simulink model "rolling_contact_36_example"  (R2026b)
settings: Solver=VariableStepAuto  StopTime=5
undefined symbols (not defined in the file): f_rr, k_gx, k_gy, k_x, m_wheel, miu_p, miu_s, mu_slide, mu_stick, omega_rr_eps, r_wheel, sgn, v_gx_max, v_gy_max, vLimit, X, Y, Z
libraries: nesl_utility x225, sm_lib x156, simulink x146, simulink_extras x36
(part 2 of 11)

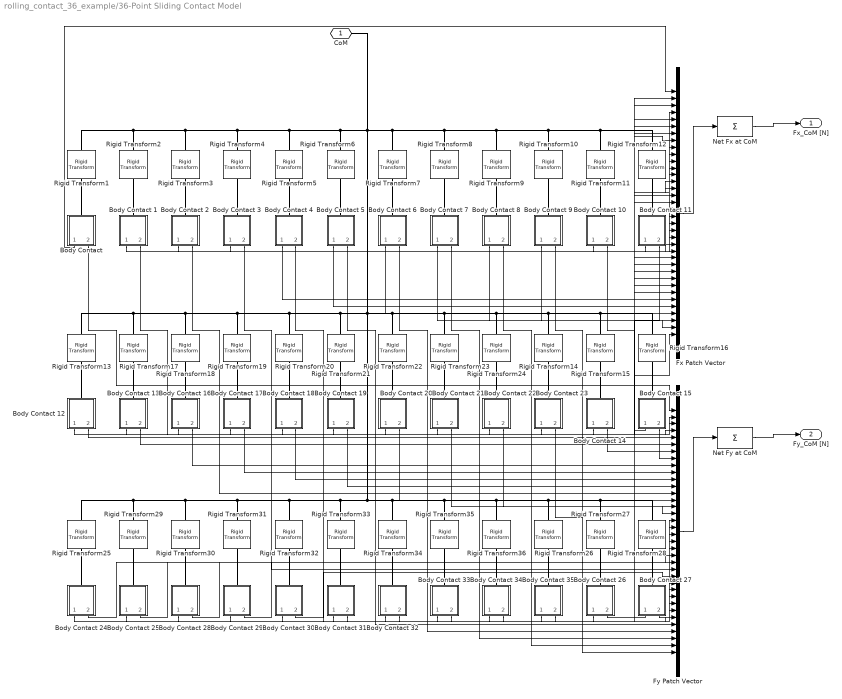
== system rolling_contact_36_example/36-Point Sliding Contact Model ==
  "Body Contact " : Subsystem
  Body Contact 1 : Subsystem
  Body Contact 10 : Subsystem
  Body Contact 11 : Subsystem
  Body Contact 12 : Subsystem
  Body Contact 13 : Subsystem
  Body Contact 14 : Subsystem
  Body Contact 15 : Subsystem
  Body Contact 16 : Subsystem
  Body Contact 17 : Subsystem
  Body Contact 18 : Subsystem
  Body Contact 19 : Subsystem
  Body Contact 2 : Subsystem
  Body Contact 20 : Subsystem
  Body Contact 21 : Subsystem
  Body Contact 22 : Subsystem
  Body Contact 23 : Subsystem
  Body Contact 24 : Subsystem
  Body Contact 25 : Subsystem
  Body Contact 26 : Subsystem
  Body Contact 27 : Subsystem
  Body Contact 28 : Subsystem
  Body Contact 29 : Subsystem
  Body Contact 3 : Subsystem
  Body Contact 30 : Subsystem
  Body Contact 31 : Subsystem
  Body Contact 32 : Subsystem
  Body Contact 33 : Subsystem
  Body Contact 34 : Subsystem
  Body Contact 35 : Subsystem
  Body Contact 4 : Subsystem
  Body Contact 5 : Subsystem
  Body Contact 6 : Subsystem
  Body Contact 7 : Subsystem
  Body Contact 8 : Subsystem
  Body Contact 9 : Subsystem
  Fx Patch Vector : Mux  Inputs=36
  Fy Patch Vector : Mux  Inputs=36
  Net Fx at CoM : Sum  Inputs=+
  Net Fy at CoM : Sum  Inputs=+
  Rigid Transform1 : sm_lib/Frames and Transforms/Rigid Transform  RotationMethod=None  FollAlignAxisA=+X  BaseAlignAxisA=+Y  FollAlignAxisB=+Y  BaseAlignAxisB=+Z  RotationStandardAxis=+Z  RotationAngle=0.0  RotationAngleUnits=deg  RotationArbitraryAxis=[0 0 1]  RotationSequenceAxes=FollowerAxes  RotationSequence=XYX  RotationSequenceAngles=[0 0 0]  RotationSequenceAnglesUnits=deg  RotationMatrix=[1 0 0; 0 1 0; 0 0 1]  Quaternion=[1 0 0 0]  TranslationMethod=Cylindrical  TranslationCartesianOffset=[0 0 0]  TranslationCartesianOffsetUnits=m  TranslationStandardAxis=+X  TranslationStandardOffset=+0.5  TranslationStandardOffsetUnits=m  TranslationROffset=r_ball  TranslationROffsetUnits=m  TranslationThetaOffset=0  TranslationThetaOffsetUnits=deg  TranslationZOffset=0  TranslationZOffsetUnits=m
  Rigid Transform10 : sm_lib/Frames and Transforms/Rigid Transform  RotationMethod=None  FollAlignAxisA=+X  BaseAlignAxisA=+Y  FollAlignAxisB=+Y  BaseAlignAxisB=+Z  RotationStandardAxis=+Z  RotationAngle=0.0  RotationAngleUnits=deg  RotationArbitraryAxis=[0 0 1]  RotationSequenceAxes=FollowerAxes  RotationSequence=XYX  RotationSequenceAngles=[0 0 0]  RotationSequenceAnglesUnits=deg  RotationMatrix=[1 0 0; 0 1 0; 0 0 1]  Quaternion=[1 0 0 0]  TranslationMethod=Cylindrical  TranslationCartesianOffset=[0 0 0]  TranslationCartesianOffsetUnits=m  TranslationStandardAxis=+X  TranslationStandardOffset=+0.5  TranslationStandardOffsetUnits=m  TranslationROffset=r_ball  TranslationROffsetUnits=m  TranslationThetaOffset=90  TranslationThetaOffsetUnits=deg  TranslationZOffset=0  TranslationZOffsetUnits=m
  Rigid Transform11 : sm_lib/Frames and Transforms/Rigid Transform  RotationMethod=None  FollAlignAxisA=+X  BaseAlignAxisA=+Y  FollAlignAxisB=+Y  BaseAlignAxisB=+Z  RotationStandardAxis=+Z  RotationAngle=0.0  RotationAngleUnits=deg  RotationArbitraryAxis=[0 0 1]  RotationSequenceAxes=FollowerAxes  RotationSequence=XYX  RotationSequenceAngles=[0 0 0]  RotationSequenceAnglesUnits=deg  RotationMatrix=[1 0 0; 0 1 0; 0 0 1]  Quaternion=[1 0 0 0]  TranslationMethod=Cylindrical  TranslationCartesianOffset=[0 0 0]  TranslationCartesianOffsetUnits=m  TranslationStandardAxis=+X  TranslationStandardOffset=+0.5  TranslationStandardOffsetUnits=m  TranslationROffset=r_ball  TranslationROffsetUnits=m  TranslationThetaOffset=100  TranslationThetaOffsetUnits=deg  TranslationZOffset=0  TranslationZOffsetUnits=m
  Rigid Transform12 : sm_lib/Frames and Transforms/Rigid Transform  RotationMethod=None  FollAlignAxisA=+X  BaseAlignAxisA=+Y  FollAlignAxisB=+Y  BaseAlignAxisB=+Z  RotationStandardAxis=+Z  RotationAngle=0.0  RotationAngleUnits=deg  RotationArbitraryAxis=[0 0 1]  RotationSequenceAxes=FollowerAxes  RotationSequence=XYX  RotationSequenceAngles=[0 0 0]  RotationSequenceAnglesUnits=deg  RotationMatrix=[1 0 0; 0 1 0; 0 0 1]  Quaternion=[1 0 0 0]  TranslationMethod=Cylindrical  TranslationCartesianOffset=[0 0 0]  TranslationCartesianOffsetUnits=m  TranslationStandardAxis=+X  TranslationStandardOffset=+0.5  TranslationStandardOffsetUnits=m  TranslationROffset=r_ball  TranslationROffsetUnits=m  TranslationThetaOffset=110  TranslationThetaOffsetUnits=deg  TranslationZOffset=0  TranslationZOffsetUnits=m
  Rigid Transform13 : sm_lib/Frames and Transforms/Rigid Transform  RotationMethod=None  FollAlignAxisA=+X  BaseAlignAxisA=+Y  FollAlignAxisB=+Y  BaseAlignAxisB=+Z  RotationStandardAxis=+Z  RotationAngle=0.0  RotationAngleUnits=deg  RotationArbitraryAxis=[0 0 1]  RotationSequenceAxes=FollowerAxes  RotationSequence=XYX  RotationSequenceAngles=[0 0 0]  RotationSequenceAnglesUnits=deg  RotationMatrix=[1 0 0; 0 1 0; 0 0 1]  Quaternion=[1 0 0 0]  TranslationMethod=Cylindrical  TranslationCartesianOffset=[0 0 0]  TranslationCartesianOffsetUnits=m  TranslationStandardAxis=+X  TranslationStandardOffset=+0.5  TranslationStandardOffsetUnits=m  TranslationROffset=r_ball  TranslationROffsetUnits=m  TranslationThetaOffset=120  TranslationThetaOffsetUnits=deg  TranslationZOffset=0  TranslationZOffsetUnits=m
  Rigid Transform14 : sm_lib/Frames and Transforms/Rigid Transform  RotationMethod=None  FollAlignAxisA=+X  BaseAlignAxisA=+Y  FollAlignAxisB=+Y  BaseAlignAxisB=+Z  RotationStandardAxis=+Z  RotationAngle=0.0  RotationAngleUnits=deg  RotationArbitraryAxis=[0 0 1]  RotationSequenceAxes=FollowerAxes  RotationSequence=XYX  RotationSequenceAngles=[0 0 0]  RotationSequenceAnglesUnits=deg  RotationMatrix=[1 0 0; 0 1 0; 0 0 1]  Quaternion=[1 0 0 0]  TranslationMethod=Cylindrical  TranslationCartesianOffset=[0 0 0]  TranslationCartesianOffsetUnits=m  TranslationStandardAxis=+X  TranslationStandardOffset=+0.5  TranslationStandardOffsetUnits=m  TranslationROffset=r_ball  TranslationROffsetUnits=m  TranslationThetaOffset=210  TranslationThetaOffsetUnits=deg  TranslationZOffset=0  TranslationZOffsetUnits=m
  Rigid Transform15 : sm_lib/Frames and Transforms/Rigid Transform  RotationMethod=None  FollAlignAxisA=+X  BaseAlignAxisA=+Y  FollAlignAxisB=+Y  BaseAlignAxisB=+Z  RotationStandardAxis=+Z  RotationAngle=0.0  RotationAngleUnits=deg  RotationArbitraryAxis=[0 0 1]  RotationSequenceAxes=FollowerAxes  RotationSequence=XYX  RotationSequenceAngles=[0 0 0]  RotationSequenceAnglesUnits=deg  RotationMatrix=[1 0 0; 0 1 0; 0 0 1]  Quaternion=[1 0 0 0]  TranslationMethod=Cylindrical  TranslationCartesianOffset=[0 0 0]  TranslationCartesianOffsetUnits=m  TranslationStandardAxis=+X  TranslationStandardOffset=+0.5  TranslationStandardOffsetUnits=m  TranslationROffset=r_ball  TranslationROffsetUnits=m  TranslationThetaOffset=220  TranslationThetaOffsetUnits=deg  TranslationZOffset=0  TranslationZOffsetUnits=m
  Rigid Transform16 : sm_lib/Frames and Transforms/Rigid Transform  RotationMethod=None  FollAlignAxisA=+X  BaseAlignAxisA=+Y  FollAlignAxisB=+Y  BaseAlignAxisB=+Z  RotationStandardAxis=+Z  RotationAngle=0.0  RotationAngleUnits=deg  RotationArbitraryAxis=[0 0 1]  RotationSequenceAxes=FollowerAxes  RotationSequence=XYX  RotationSequenceAngles=[0 0 0]  RotationSequenceAnglesUnits=deg  RotationMatrix=[1 0 0; 0 1 0; 0 0 1]  Quaternion=[1 0 0 0]  TranslationMethod=Cylindrical  TranslationCartesianOffset=[0 0 0]  TranslationCartesianOffsetUnits=m  TranslationStandardAxis=+X  TranslationStandardOffset=+0.5  TranslationStandardOffsetUnits=m  TranslationROffset=r_ball  TranslationROffsetUnits=m  TranslationThetaOffset=230  TranslationThetaOffsetUnits=deg  TranslationZOffset=0  TranslationZOffsetUnits=m
  Rigid Transform17 : sm_lib/Frames and Transforms/Rigid Transform  RotationMethod=None  FollAlignAxisA=+X  BaseAlignAxisA=+Y  FollAlignAxisB=+Y  BaseAlignAxisB=+Z  RotationStandardAxis=+Z  RotationAngle=0.0  RotationAngleUnits=deg  RotationArbitraryAxis=[0 0 1]  RotationSequenceAxes=FollowerAxes  RotationSequence=XYX  RotationSequenceAngles=[0 0 0]  RotationSequenceAnglesUnits=deg  RotationMatrix=[1 0 0; 0 1 0; 0 0 1]  Quaternion=[1 0 0 0]  TranslationMethod=Cylindrical  TranslationCartesianOffset=[0 0 0]  TranslationCartesianOffsetUnits=m  TranslationStandardAxis=+X  TranslationStandardOffset=+0.5  TranslationStandardOffsetUnits=m  TranslationROffset=r_ball  TranslationROffsetUnits=m  TranslationThetaOffset=130  TranslationThetaOffsetUnits=deg  TranslationZOffset=0  TranslationZOffsetUnits=m
  Rigid Transform18 : sm_lib/Frames and Transforms/Rigid Transform  RotationMethod=None  FollAlignAxisA=+X  BaseAlignAxisA=+Y  FollAlignAxisB=+Y  BaseAlignAxisB=+Z  RotationStandardAxis=+Z  RotationAngle=0.0  RotationAngleUnits=deg  RotationArbitraryAxis=[0 0 1]  RotationSequenceAxes=FollowerAxes  RotationSequence=XYX  RotationSequenceAngles=[0 0 0]  RotationSequenceAnglesUnits=deg  RotationMatrix=[1 0 0; 0 1 0; 0 0 1]  Quaternion=[1 0 0 0]  TranslationMethod=Cylindrical  TranslationCartesianOffset=[0 0 0]  TranslationCartesianOffsetUnits=m  TranslationStandardAxis=+X  TranslationStandardOffset=+0.5  TranslationStandardOffsetUnits=m  TranslationROffset=r_ball  TranslationROffsetUnits=m  TranslationThetaOffset=140  TranslationThetaOffsetUnits=deg  TranslationZOffset=0  TranslationZOffsetUnits=m
  Rigid Transform19 : sm_lib/Frames and Transforms/Rigid Transform  RotationMethod=None  FollAlignAxisA=+X  BaseAlignAxisA=+Y  FollAlignAxisB=+Y  BaseAlignAxisB=+Z  RotationStandardAxis=+Z  RotationAngle=0.0  RotationAngleUnits=deg  RotationArbitraryAxis=[0 0 1]  RotationSequenceAxes=FollowerAxes  RotationSequence=XYX  RotationSequenceAngles=[0 0 0]  RotationSequenceAnglesUnits=deg  RotationMatrix=[1 0 0; 0 1 0; 0 0 1]  Quaternion=[1 0 0 0]  TranslationMethod=Cylindrical  TranslationCartesianOffset=[0 0 0]  TranslationCartesianOffsetUnits=m  TranslationStandardAxis=+X  TranslationStandardOffset=+0.5  TranslationStandardOffsetUnits=m  TranslationROffset=r_ball  TranslationROffsetUnits=m  TranslationThetaOffset=150  TranslationThetaOffsetUnits=deg  TranslationZOffset=0  TranslationZOffsetUnits=m
  Rigid Transform2 : sm_lib/Frames and Transforms/Rigid Transform  RotationMethod=None  FollAlignAxisA=+X  BaseAlignAxisA=+Y  FollAlignAxisB=+Y  BaseAlignAxisB=+Z  RotationStandardAxis=+Z  RotationAngle=0.0  RotationAngleUnits=deg  RotationArbitraryAxis=[0 0 1]  RotationSequenceAxes=FollowerAxes  RotationSequence=XYX  RotationSequenceAngles=[0 0 0]  RotationSequenceAnglesUnits=deg  RotationMatrix=[1 0 0; 0 1 0; 0 0 1]  Quaternion=[1 0 0 0]  TranslationMethod=Cylindrical  TranslationCartesianOffset=[0 0 0]  TranslationCartesianOffsetUnits=m  TranslationStandardAxis=+X  TranslationStandardOffset=+0.5  TranslationStandardOffsetUnits=m  TranslationROffset=r_ball  TranslationROffsetUnits=m  TranslationThetaOffset=10  TranslationThetaOffsetUnits=deg  TranslationZOffset=0  TranslationZOffsetUnits=m
  Rigid Transform20 : sm_lib/Frames and Transforms/Rigid Transform  RotationMethod=None  FollAlignAxisA=+X  BaseAlignAxisA=+Y  FollAlignAxisB=+Y  BaseAlignAxisB=+Z  RotationStandardAxis=+Z  RotationAngle=0.0  RotationAngleUnits=deg  RotationArbitraryAxis=[0 0 1]  RotationSequenceAxes=FollowerAxes  RotationSequence=XYX  RotationSequenceAngles=[0 0 0]  RotationSequenceAnglesUnits=deg  RotationMatrix=[1 0 0; 0 1 0; 0 0 1]  Quaternion=[1 0 0 0]  TranslationMethod=Cylindrical  TranslationCartesianOffset=[0 0 0]  TranslationCartesianOffsetUnits=m  TranslationStandardAxis=+X  TranslationStandardOffset=+0.5  TranslationStandardOffsetUnits=m  TranslationROffset=r_ball  TranslationROffsetUnits=m  TranslationThetaOffset=160  TranslationThetaOffsetUnits=deg  TranslationZOffset=0  TranslationZOffsetUnits=m
  Rigid Transform21 : sm_lib/Frames and Transforms/Rigid Transform  RotationMethod=None  FollAlignAxisA=+X  BaseAlignAxisA=+Y  FollAlignAxisB=+Y  BaseAlignAxisB=+Z  RotationStandardAxis=+Z  RotationAngle=0.0  RotationAngleUnits=deg  RotationArbitraryAxis=[0 0 1]  RotationSequenceAxes=FollowerAxes  RotationSequence=XYX  RotationSequenceAngles=[0 0 0]  RotationSequenceAnglesUnits=deg  RotationMatrix=[1 0 0; 0 1 0; 0 0 1]  Quaternion=[1 0 0 0]  TranslationMethod=Cylindrical  TranslationCartesianOffset=[0 0 0]  TranslationCartesianOffsetUnits=m  TranslationStandardAxis=+X  TranslationStandardOffset=+0.5  TranslationStandardOffsetUnits=m  TranslationROffset=r_ball  TranslationROffsetUnits=m  TranslationThetaOffset=170  TranslationThetaOffsetUnits=deg  TranslationZOffset=0  TranslationZOffsetUnits=m
  Rigid Transform22 : sm_lib/Frames and Transforms/Rigid Transform  RotationMethod=None  FollAlignAxisA=+X  BaseAlignAxisA=+Y  FollAlignAxisB=+Y  BaseAlignAxisB=+Z  RotationStandardAxis=+Z  RotationAngle=0.0  RotationAngleUnits=deg  RotationArbitraryAxis=[0 0 1]  RotationSequenceAxes=FollowerAxes  RotationSequence=XYX  RotationSequenceAngles=[0 0 0]  RotationSequenceAnglesUnits=deg  RotationMatrix=[1 0 0; 0 1 0; 0 0 1]  Quaternion=[1 0 0 0]  TranslationMethod=Cylindrical  TranslationCartesianOffset=[0 0 0]  TranslationCartesianOffsetUnits=m  TranslationStandardAxis=+X  TranslationStandardOffset=+0.5  TranslationStandardOffsetUnits=m  TranslationROffset=r_ball  TranslationROffsetUnits=m  TranslationThetaOffset=180  TranslationThetaOffsetUnits=deg  TranslationZOffset=0  TranslationZOffsetUnits=m
  Rigid Transform23 : sm_lib/Frames and Transforms/Rigid Transform  RotationMethod=None  FollAlignAxisA=+X  BaseAlignAxisA=+Y  FollAlignAxisB=+Y  BaseAlignAxisB=+Z  RotationStandardAxis=+Z  RotationAngle=0.0  RotationAngleUnits=deg  RotationArbitraryAxis=[0 0 1]  RotationSequenceAxes=FollowerAxes  RotationSequence=XYX  RotationSequenceAngles=[0 0 0]  RotationSequenceAnglesUnits=deg  RotationMatrix=[1 0 0; 0 1 0; 0 0 1]  Quaternion=[1 0 0 0]  TranslationMethod=Cylindrical  TranslationCartesianOffset=[0 0 0]  TranslationCartesianOffsetUnits=m  TranslationStandardAxis=+X  TranslationStandardOffset=+0.5  TranslationStandardOffsetUnits=m  TranslationROffset=r_ball  TranslationROffsetUnits=m  TranslationThetaOffset=190  TranslationThetaOffsetUnits=deg  TranslationZOffset=0  TranslationZOffsetUnits=m
  Rigid Transform24 : sm_lib/Frames and Transforms/Rigid Transform  RotationMethod=None  FollAlignAxisA=+X  BaseAlignAxisA=+Y  FollAlignAxisB=+Y  BaseAlignAxisB=+Z  RotationStandardAxis=+Z  RotationAngle=0.0  RotationAngleUnits=deg  RotationArbitraryAxis=[0 0 1]  RotationSequenceAxes=FollowerAxes  RotationSequence=XYX  RotationSequenceAngles=[0 0 0]  RotationSequenceAnglesUnits=deg  RotationMatrix=[1 0 0; 0 1 0; 0 0 1]  Quaternion=[1 0 0 0]  TranslationMethod=Cylindrical  TranslationCartesianOffset=[0 0 0]  TranslationCartesianOffsetUnits=m  TranslationStandardAxis=+X  TranslationStandardOffset=+0.5  TranslationStandardOffsetUnits=m  TranslationROffset=r_ball  TranslationROffsetUnits=m  TranslationThetaOffset=200  TranslationThetaOffsetUnits=deg  TranslationZOffset=0  TranslationZOffsetUnits=m
  Rigid Transform25 : sm_lib/Frames and Transforms/Rigid Transform  RotationMethod=None  FollAlignAxisA=+X  BaseAlignAxisA=+Y  FollAlignAxisB=+Y  BaseAlignAxisB=+Z  RotationStandardAxis=+Z  RotationAngle=0.0  RotationAngleUnits=deg  RotationArbitraryAxis=[0 0 1]  RotationSequenceAxes=FollowerAxes  RotationSequence=XYX  RotationSequenceAngles=[0 0 0]  RotationSequenceAnglesUnits=deg  RotationMatrix=[1 0 0; 0 1 0; 0 0 1]  Quaternion=[1 0 0 0]  TranslationMethod=Cylindrical  TranslationCartesianOffset=[0 0 0]  TranslationCartesianOffsetUnits=m  TranslationStandardAxis=+X  TranslationStandardOffset=+0.5  TranslationStandardOffsetUnits=m  TranslationROffset=r_ball  TranslationROffsetUnits=m  TranslationThetaOffset=240  TranslationThetaOffsetUnits=deg  TranslationZOffset=0  TranslationZOffsetUnits=m
  Rigid Transform26 : sm_lib/Frames and Transforms/Rigid Transform  RotationMethod=None  FollAlignAxisA=+X  BaseAlignAxisA=+Y  FollAlignAxisB=+Y  BaseAlignAxisB=+Z  RotationStandardAxis=+Z  RotationAngle=0.0  RotationAngleUnits=deg  RotationArbitraryAxis=[0 0 1]  RotationSequenceAxes=FollowerAxes  RotationSequence=XYX  RotationSequenceAngles=[0 0 0]  RotationSequenceAnglesUnits=deg  RotationMatrix=[1 0 0; 0 1 0; 0 0 1]  Quaternion=[1 0 0 0]  TranslationMethod=Cylindrical  TranslationCartesianOffset=[0 0 0]  TranslationCartesianOffsetUnits=m  TranslationStandardAxis=+X  TranslationStandardOffset=+0.5  TranslationStandardOffsetUnits=m  TranslationROffset=r_ball  TranslationROffsetUnits=m  TranslationThetaOffset=330  TranslationThetaOffsetUnits=deg  TranslationZOffset=0  TranslationZOffsetUnits=m
  Rigid Transform27 : sm_lib/Frames and Transforms/Rigid Transform  RotationMethod=None  FollAlignAxisA=+X  BaseAlignAxisA=+Y  FollAlignAxisB=+Y  BaseAlignAxisB=+Z  RotationStandardAxis=+Z  RotationAngle=0.0  RotationAngleUnits=deg  RotationArbitraryAxis=[0 0 1]  RotationSequenceAxes=FollowerAxes  RotationSequence=XYX  RotationSequenceAngles=[0 0 0]  RotationSequenceAnglesUnits=deg  RotationMatrix=[1 0 0; 0 1 0; 0 0 1]  Quaternion=[1 0 0 0]  TranslationMethod=Cylindrical  TranslationCartesianOffset=[0 0 0]  TranslationCartesianOffsetUnits=m  TranslationStandardAxis=+X  TranslationStandardOffset=+0.5  TranslationStandardOffsetUnits=m  TranslationROffset=r_ball  TranslationROffsetUnits=m  TranslationThetaOffset=340  TranslationThetaOffsetUnits=deg  TranslationZOffset=0  TranslationZOffsetUnits=m
  Rigid Transform28 : sm_lib/Frames and Transforms/Rigid Transform  RotationMethod=None  FollAlignAxisA=+X  BaseAlignAxisA=+Y  FollAlignAxisB=+Y  BaseAlignAxisB=+Z  RotationStandardAxis=+Z  RotationAngle=0.0  RotationAngleUnits=deg  RotationArbitraryAxis=[0 0 1]  RotationSequenceAxes=FollowerAxes  RotationSequence=XYX  RotationSequenceAngles=[0 0 0]  RotationSequenceAnglesUnits=deg  RotationMatrix=[1 0 0; 0 1 0; 0 0 1]  Quaternion=[1 0 0 0]  TranslationMethod=Cylindrical  TranslationCartesianOffset=[0 0 0]  TranslationCartesianOffsetUnits=m  TranslationStandardAxis=+X  TranslationStandardOffset=+0.5  TranslationStandardOffsetUnits=m  TranslationROffset=r_ball  TranslationROffsetUnits=m  TranslationThetaOffset=350  TranslationThetaOffsetUnits=deg  TranslationZOffset=0  TranslationZOffsetUnits=m
  Rigid Transform29 : sm_lib/Frames and Transforms/Rigid Transform  RotationMethod=None  FollAlignAxisA=+X  BaseAlignAxisA=+Y  FollAlignAxisB=+Y  BaseAlignAxisB=+Z  RotationStandardAxis=+Z  RotationAngle=0.0  RotationAngleUnits=deg  RotationArbitraryAxis=[0 0 1]  RotationSequenceAxes=FollowerAxes  RotationSequence=XYX  RotationSequenceAngles=[0 0 0]  RotationSequenceAnglesUnits=deg  RotationMatrix=[1 0 0; 0 1 0; 0 0 1]  Quaternion=[1 0 0 0]  TranslationMethod=Cylindrical  TranslationCartesianOffset=[0 0 0]  TranslationCartesianOffsetUnits=m  TranslationStandardAxis=+X  TranslationStandardOffset=+0.5  TranslationStandardOffsetUnits=m  TranslationROffset=r_ball  TranslationROffsetUnits=m  TranslationThetaOffset=250  TranslationThetaOffsetUnits=deg  TranslationZOffset=0  TranslationZOffsetUnits=m
  Rigid Transform3 : sm_lib/Frames and Transforms/Rigid Transform  RotationMethod=None  FollAlignAxisA=+X  BaseAlignAxisA=+Y  FollAlignAxisB=+Y  BaseAlignAxisB=+Z  RotationStandardAxis=+Z  RotationAngle=0.0  RotationAngleUnits=deg  RotationArbitraryAxis=[0 0 1]  RotationSequenceAxes=FollowerAxes  RotationSequence=XYX  RotationSequenceAngles=[0 0 0]  RotationSequenceAnglesUnits=deg  RotationMatrix=[1 0 0; 0 1 0; 0 0 1]  Quaternion=[1 0 0 0]  TranslationMethod=Cylindrical  TranslationCartesianOffset=[0 0 0]  TranslationCartesianOffsetUnits=m  TranslationStandardAxis=+X  TranslationStandardOffset=+0.5  TranslationStandardOffsetUnits=m  TranslationROffset=r_ball  TranslationROffsetUnits=m  TranslationThetaOffset=20  TranslationThetaOffsetUnits=deg  TranslationZOffset=0  TranslationZOffsetUnits=m
  Rigid Transform30 : sm_lib/Frames and Transforms/Rigid Transform  RotationMethod=None  FollAlignAxisA=+X  BaseAlignAxisA=+Y  FollAlignAxisB=+Y  BaseAlignAxisB=+Z  RotationStandardAxis=+Z  RotationAngle=0.0  RotationAngleUnits=deg  RotationArbitraryAxis=[0 0 1]  RotationSequenceAxes=FollowerAxes  RotationSequence=XYX  RotationSequenceAngles=[0 0 0]  RotationSequenceAnglesUnits=deg  RotationMatrix=[1 0 0; 0 1 0; 0 0 1]  Quaternion=[1 0 0 0]  TranslationMethod=Cylindrical  TranslationCartesianOffset=[0 0 0]  TranslationCartesianOffsetUnits=m  TranslationStandardAxis=+X  TranslationStandardOffset=+0.5  TranslationStandardOffsetUnits=m  TranslationROffset=r_ball  TranslationROffsetUnits=m  TranslationThetaOffset=260  TranslationThetaOffsetUnits=deg  TranslationZOffset=0  TranslationZOffsetUnits=m
  Rigid Transform31 : sm_lib/Frames and Transforms/Rigid Transform  RotationMethod=None  FollAlignAxisA=+X  BaseAlignAxisA=+Y  FollAlignAxisB=+Y  BaseAlignAxisB=+Z  RotationStandardAxis=+Z  RotationAngle=0.0  RotationAngleUnits=deg  RotationArbitraryAxis=[0 0 1]  RotationSequenceAxes=FollowerAxes  RotationSequence=XYX  RotationSequenceAngles=[0 0 0]  RotationSequenceAnglesUnits=deg  RotationMatrix=[1 0 0; 0 1 0; 0 0 1]  Quaternion=[1 0 0 0]  TranslationMethod=Cylindrical  TranslationCartesianOffset=[0 0 0]  TranslationCartesianOffsetUnits=m  TranslationStandardAxis=+X  TranslationStandardOffset=+0.5  TranslationStandardOffsetUnits=m  TranslationROffset=r_ball  TranslationROffsetUnits=m  TranslationThetaOffset=270  TranslationThetaOffsetUnits=deg  TranslationZOffset=0  TranslationZOffsetUnits=m
  Rigid Transform32 : sm_lib/Frames and Transforms/Rigid Transform  RotationMethod=None  FollAlignAxisA=+X  BaseAlignAxisA=+Y  FollAlignAxisB=+Y  BaseAlignAxisB=+Z  RotationStandardAxis=+Z  RotationAngle=0.0  RotationAngleUnits=deg  RotationArbitraryAxis=[0 0 1]  RotationSequenceAxes=FollowerAxes  RotationSequence=XYX  RotationSequenceAngles=[0 0 0]  RotationSequenceAnglesUnits=deg  RotationMatrix=[1 0 0; 0 1 0; 0 0 1]  Quaternion=[1 0 0 0]  TranslationMethod=Cylindrical  TranslationCartesianOffset=[0 0 0]  TranslationCartesianOffsetUnits=m  TranslationStandardAxis=+X  TranslationStandardOffset=+0.5  TranslationStandardOffsetUnits=m  TranslationROffset=r_ball  TranslationROffsetUnits=m  TranslationThetaOffset=280  TranslationThetaOffsetUnits=deg  TranslationZOffset=0  TranslationZOffsetUnits=m
  Rigid Transform33 : sm_lib/Frames and Transforms/Rigid Transform  RotationMethod=None  FollAlignAxisA=+X  BaseAlignAxisA=+Y  FollAlignAxisB=+Y  BaseAlignAxisB=+Z  RotationStandardAxis=+Z  RotationAngle=0.0  RotationAngleUnits=deg  RotationArbitraryAxis=[0 0 1]  RotationSequenceAxes=FollowerAxes  RotationSequence=XYX  RotationSequenceAngles=[0 0 0]  RotationSequenceAnglesUnits=deg  RotationMatrix=[1 0 0; 0 1 0; 0 0 1]  Quaternion=[1 0 0 0]  TranslationMethod=Cylindrical  TranslationCartesianOffset=[0 0 0]  TranslationCartesianOffsetUnits=m  TranslationStandardAxis=+X  TranslationStandardOffset=+0.5  TranslationStandardOffsetUnits=m  TranslationROffset=r_ball  TranslationROffsetUnits=m  TranslationThetaOffset=290  TranslationThetaOffsetUnits=deg  TranslationZOffset=0  TranslationZOffsetUnits=m
  Rigid Transform34 : sm_lib/Frames and Transforms/Rigid Transform  RotationMethod=None  FollAlignAxisA=+X  BaseAlignAxisA=+Y  FollAlignAxisB=+Y  BaseAlignAxisB=+Z  RotationStandardAxis=+Z  RotationAngle=0.0  RotationAngleUnits=deg  RotationArbitraryAxis=[0 0 1]  RotationSequenceAxes=FollowerAxes  RotationSequence=XYX  RotationSequenceAngles=[0 0 0]  RotationSequenceAnglesUnits=deg  RotationMatrix=[1 0 0; 0 1 0; 0 0 1]  Quaternion=[1 0 0 0]  TranslationMethod=Cylindrical  TranslationCartesianOffset=[0 0 0]  TranslationCartesianOffsetUnits=m  TranslationStandardAxis=+X  TranslationStandardOffset=+0.5  TranslationStandardOffsetUnits=m  TranslationROffset=r_ball  TranslationROffsetUnits=m  TranslationThetaOffset=300  TranslationThetaOffsetUnits=deg  TranslationZOffset=0  TranslationZOffsetUnits=m
  Rigid Transform35 : sm_lib/Frames and Transforms/Rigid Transform  RotationMethod=None  FollAlignAxisA=+X  BaseAlignAxisA=+Y  FollAlignAxisB=+Y  BaseAlignAxisB=+Z  RotationStandardAxis=+Z  RotationAngle=0.0  RotationAngleUnits=deg  RotationArbitraryAxis=[0 0 1]  RotationSequenceAxes=FollowerAxes  RotationSequence=XYX  RotationSequenceAngles=[0 0 0]  RotationSequenceAnglesUnits=deg  RotationMatrix=[1 0 0; 0 1 0; 0 0 1]  Quaternion=[1 0 0 0]  TranslationMethod=Cylindrical  TranslationCartesianOffset=[0 0 0]  TranslationCartesianOffsetUnits=m  TranslationStandardAxis=+X  TranslationStandardOffset=+0.5  TranslationStandardOffsetUnits=m  TranslationROffset=r_ball  TranslationROffsetUnits=m  TranslationThetaOffset=310  TranslationThetaOffsetUnits=deg  TranslationZOffset=0  TranslationZOffsetUnits=m
  Rigid Transform36 : sm_lib/Frames and Transforms/Rigid Transform  RotationMethod=None  FollAlignAxisA=+X  BaseAlignAxisA=+Y  FollAlignAxisB=+Y  BaseAlignAxisB=+Z  RotationStandardAxis=+Z  RotationAngle=0.0  RotationAngleUnits=deg  RotationArbitraryAxis=[0 0 1]  RotationSequenceAxes=FollowerAxes  RotationSequence=XYX  RotationSequenceAngles=[0 0 0]  RotationSequenceAnglesUnits=deg  RotationMatrix=[1 0 0; 0 1 0; 0 0 1]  Quaternion=[1 0 0 0]  TranslationMethod=Cylindrical  TranslationCartesianOffset=[0 0 0]  TranslationCartesianOffsetUnits=m  TranslationStandardAxis=+X  TranslationStandardOffset=+0.5  TranslationStandardOffsetUnits=m  TranslationROffset=r_ball  TranslationROffsetUnits=m  TranslationThetaOffset=320  TranslationThetaOffsetUnits=deg  TranslationZOffset=0  TranslationZOffsetUnits=m
  Rigid Transform4 : sm_lib/Frames and Transforms/Rigid Transform  RotationMethod=None  FollAlignAxisA=+X  BaseAlignAxisA=+Y  FollAlignAxisB=+Y  BaseAlignAxisB=+Z  RotationStandardAxis=+Z  RotationAngle=0.0  RotationAngleUnits=deg  RotationArbitraryAxis=[0 0 1]  RotationSequenceAxes=FollowerAxes  RotationSequence=XYX  RotationSequenceAngles=[0 0 0]  RotationSequenceAnglesUnits=deg  RotationMatrix=[1 0 0; 0 1 0; 0 0 1]  Quaternion=[1 0 0 0]  TranslationMethod=Cylindrical  TranslationCartesianOffset=[0 0 0]  TranslationCartesianOffsetUnits=m  TranslationStandardAxis=+X  TranslationStandardOffset=+0.5  TranslationStandardOffsetUnits=m  TranslationROffset=r_ball  TranslationROffsetUnits=m  TranslationThetaOffset=30  TranslationThetaOffsetUnits=deg  TranslationZOffset=0  TranslationZOffsetUnits=m
  Rigid Transform5 : sm_lib/Frames and Transforms/Rigid Transform  RotationMethod=None  FollAlignAxisA=+X  BaseAlignAxisA=+Y  FollAlignAxisB=+Y  BaseAlignAxisB=+Z  RotationStandardAxis=+Z  RotationAngle=0.0  RotationAngleUnits=deg  RotationArbitraryAxis=[0 0 1]  RotationSequenceAxes=FollowerAxes  RotationSequence=XYX  RotationSequenceAngles=[0 0 0]  RotationSequenceAnglesUnits=deg  RotationMatrix=[1 0 0; 0 1 0; 0 0 1]  Quaternion=[1 0 0 0]  TranslationMethod=Cylindrical  TranslationCartesianOffset=[0 0 0]  TranslationCartesianOffsetUnits=m  TranslationStandardAxis=+X  TranslationStandardOffset=+0.5  TranslationStandardOffsetUnits=m  TranslationROffset=r_ball  TranslationROffsetUnits=m  TranslationThetaOffset=40  TranslationThetaOffsetUnits=deg  TranslationZOffset=0  TranslationZOffsetUnits=m
  Rigid Transform6 : sm_lib/Frames and Transforms/Rigid Transform  RotationMethod=None  FollAlignAxisA=+X  BaseAlignAxisA=+Y  FollAlignAxisB=+Y  BaseAlignAxisB=+Z  RotationStandardAxis=+Z  RotationAngle=0.0  RotationAngleUnits=deg  RotationArbitraryAxis=[0 0 1]  RotationSequenceAxes=FollowerAxes  RotationSequence=XYX  RotationSequenceAngles=[0 0 0]  RotationSequenceAnglesUnits=deg  RotationMatrix=[1 0 0; 0 1 0; 0 0 1]  Quaternion=[1 0 0 0]  TranslationMethod=Cylindrical  TranslationCartesianOffset=[0 0 0]  TranslationCartesianOffsetUnits=m  TranslationStandardAxis=+X  TranslationStandardOffset=+0.5  TranslationStandardOffsetUnits=m  TranslationROffset=r_ball  TranslationROffsetUnits=m  TranslationThetaOffset=50  TranslationThetaOffsetUnits=deg  TranslationZOffset=0  TranslationZOffsetUnits=m
  Rigid Transform7 : sm_lib/Frames and Transforms/Rigid Transform  RotationMethod=None  FollAlignAxisA=+X  BaseAlignAxisA=+Y  FollAlignAxisB=+Y  BaseAlignAxisB=+Z  RotationStandardAxis=+Z  RotationAngle=0.0  RotationAngleUnits=deg  RotationArbitraryAxis=[0 0 1]  RotationSequenceAxes=FollowerAxes  RotationSequence=XYX  RotationSequenceAngles=[0 0 0]  RotationSequenceAnglesUnits=deg  RotationMatrix=[1 0 0; 0 1 0; 0 0 1]  Quaternion=[1 0 0 0]  TranslationMethod=Cylindrical  TranslationCartesianOffset=[0 0 0]  TranslationCartesianOffsetUnits=m  TranslationStandardAxis=+X  TranslationStandardOffset=+0.5  TranslationStandardOffsetUnits=m  TranslationROffset=r_ball  TranslationROffsetUnits=m  TranslationThetaOffset=60  TranslationThetaOffsetUnits=deg  TranslationZOffset=0  TranslationZOffsetUnits=m
  Rigid Transform8 : sm_lib/Frames and Transforms/Rigid Transform  RotationMethod=None  FollAlignAxisA=+X  BaseAlignAxisA=+Y  FollAlignAxisB=+Y  BaseAlignAxisB=+Z  RotationStandardAxis=+Z  RotationAngle=0.0  RotationAngleUnits=deg  RotationArbitraryAxis=[0 0 1]  RotationSequenceAxes=FollowerAxes  RotationSequence=XYX  RotationSequenceAngles=[0 0 0]  RotationSequenceAnglesUnits=deg  RotationMatrix=[1 0 0; 0 1 0; 0 0 1]  Quaternion=[1 0 0 0]  TranslationMethod=Cylindrical  TranslationCartesianOffset=[0 0 0]  TranslationCartesianOffsetUnits=m  TranslationStandardAxis=+X  TranslationStandardOffset=+0.5  TranslationStandardOffsetUnits=m  TranslationROffset=r_ball  TranslationROffsetUnits=m  TranslationThetaOffset=70  TranslationThetaOffsetUnits=deg  TranslationZOffset=0  TranslationZOffsetUnits=m
  Rigid Transform9 : sm_lib/Frames and Transforms/Rigid Transform  RotationMethod=None  FollAlignAxisA=+X  BaseAlignAxisA=+Y  FollAlignAxisB=+Y  BaseAlignAxisB=+Z  RotationStandardAxis=+Z  RotationAngle=0.0  RotationAngleUnits=deg  RotationArbitraryAxis=[0 0 1]  RotationSequenceAxes=FollowerAxes  RotationSequence=XYX  RotationSequenceAngles=[0 0 0]  RotationSequenceAnglesUnits=deg  RotationMatrix=[1 0 0; 0 1 0; 0 0 1]  Quaternion=[1 0 0 0]  TranslationMethod=Cylindrical  TranslationCartesianOffset=[0 0 0]  TranslationCartesianOffsetUnits=m  TranslationStandardAxis=+X  TranslationStandardOffset=+0.5  TranslationStandardOffsetUnits=m  TranslationROffset=r_ball  TranslationROffsetUnits=m  TranslationThetaOffset=80  TranslationThetaOffsetUnits=deg  TranslationZOffset=0  TranslationZOffsetUnits=m
  CoM : PMIOPort  Side=Left
  Fx_CoM [N] : Outport
  Fy_CoM [N] : Outport  Port=2
  wires:
  "Body Contact "/1(Fx patch [N]) -> Fx Patch Vector/1
  "Body Contact "/2(Fy patch [N]) -> Fy Patch Vector/1
  Body Contact 1/1(Fx patch [N]) -> Fx Patch Vector/2
  Body Contact 1/2(Fy patch [N]) -> Fy Patch Vector/2
  Body Contact 10/1(Fx patch [N]) -> Fx Patch Vector/3
  Body Contact 10/2(Fy patch [N]) -> Fy Patch Vector/3
  Body Contact 11/1(Fx patch [N]) -> Fx Patch Vector/4
  Body Contact 11/2(Fy patch [N]) -> Fy Patch Vector/4
  Body Contact 12/1(Fx patch [N]) -> Fx Patch Vector/5
  Body Contact 12/2(Fy patch [N]) -> Fy Patch Vector/5
  Body Contact 13/1(Fx patch [N]) -> Fx Patch Vector/6
  Body Contact 13/2(Fy patch [N]) -> Fy Patch Vector/6
  Body Contact 14/1(Fx patch [N]) -> Fx Patch Vector/7
  Body Contact 14/2(Fy patch [N]) -> Fy Patch Vector/7
  Body Contact 15/1(Fx patch [N]) -> Fx Patch Vector/8
  Body Contact 15/2(Fy patch [N]) -> Fy Patch Vector/8
  Body Contact 16/1(Fx patch [N]) -> Fx Patch Vector/9
  Body Contact 16/2(Fy patch [N]) -> Fy Patch Vector/9
  Body Contact 17/1(Fx patch [N]) -> Fx Patch Vector/10
  Body Contact 17/2(Fy patch [N]) -> Fy Patch Vector/10
  Body Contact 18/1(Fx patch [N]) -> Fx Patch Vector/11
  Body Contact 18/2(Fy patch [N]) -> Fy Patch Vector/11
  Body Contact 19/1(Fx patch [N]) -> Fx Patch Vector/12
  Body Contact 19/2(Fy patch [N]) -> Fy Patch Vector/12
  Body Contact 2/1(Fx patch [N]) -> Fx Patch Vector/13
  Body Contact 2/2(Fy patch [N]) -> Fy Patch Vector/13
  Body Contact 20/1(Fx patch [N]) -> Fx Patch Vector/14
  Body Contact 20/2(Fy patch [N]) -> Fy Patch Vector/14
  Body Contact 21/1(Fx patch [N]) -> Fx Patch Vector/15
  Body Contact 21/2(Fy patch [N]) -> Fy Patch Vector/15
  Body Contact 22/1(Fx patch [N]) -> Fx Patch Vector/16
  Body Contact 22/2(Fy patch [N]) -> Fy Patch Vector/16
  Body Contact 23/1(Fx patch [N]) -> Fx Patch Vector/17
  Body Contact 23/2(Fy patch [N]) -> Fy Patch Vector/17
  Body Contact 24/1(Fx patch [N]) -> Fx Patch Vector/18
  Body Contact 24/2(Fy patch [N]) -> Fy Patch Vector/18
  Body Contact 25/1(Fx patch [N]) -> Fx Patch Vector/19
  Body Contact 25/2(Fy patch [N]) -> Fy Patch Vector/19
  Body Contact 26/1(Fx patch [N]) -> Fx Patch Vector/20
  Body Contact 26/2(Fy patch [N]) -> Fy Patch Vector/20
  Body Contact 27/1(Fx patch [N]) -> Fx Patch Vector/21
  Body Contact 27/2(Fy patch [N]) -> Fy Patch Vector/21
  Body Contact 28/1(Fx patch [N]) -> Fx Patch Vector/22
  Body Contact 28/2(Fy patch [N]) -> Fy Patch Vector/22
  Body Contact 29/1(Fx patch [N]) -> Fx Patch Vector/23
  Body Contact 29/2(Fy patch [N]) -> Fy Patch Vector/23
  Body Contact 3/1(Fx patch [N]) -> Fx Patch Vector/24
  Body Contact 3/2(Fy patch [N]) -> Fy Patch Vector/24
  Body Contact 30/1(Fx patch [N]) -> Fx Patch Vector/25
  Body Contact 30/2(Fy patch [N]) -> Fy Patch Vector/25
  Body Contact 31/1(Fx patch [N]) -> Fx Patch Vector/26
  Body Contact 31/2(Fy patch [N]) -> Fy Patch Vector/26
  Body Contact 32/1(Fx patch [N]) -> Fx Patch Vector/27
  Body Contact 32/2(Fy patch [N]) -> Fy Patch Vector/27
  Body Contact 33/1(Fx patch [N]) -> Fx Patch Vector/28
  Body Contact 33/2(Fy patch [N]) -> Fy Patch Vector/28
  Body Contact 34/1(Fx patch [N]) -> Fx Patch Vector/29
  Body Contact 34/2(Fy patch [N]) -> Fy Patch Vector/29
  Body Contact 35/1(Fx patch [N]) -> Fx Patch Vector/30
  Body Contact 35/2(Fy patch [N]) -> Fy Patch Vector/30
  Body Contact 4/1(Fx patch [N]) -> Fx Patch Vector/31
  Body Contact 4/2(Fy patch [N]) -> Fy Patch Vector/31
  Body Contact 5/1(Fx patch [N]) -> Fx Patch Vector/32
  Body Contact 5/2(Fy patch [N]) -> Fy Patch Vector/32
  Body Contact 6/1(Fx patch [N]) -> Fx Patch Vector/33
  Body Contact 6/2(Fy patch [N]) -> Fy Patch Vector/33
  Body Contact 7/1(Fx patch [N]) -> Fx Patch Vector/34
  Body Contact 7/2(Fy patch [N]) -> Fy Patch Vector/34
  Body Contact 8/1(Fx patch [N]) -> Fx Patch Vector/35
  Body Contact 8/2(Fy patch [N]) -> Fy Patch Vector/35
  Body Contact 9/1(Fx patch [N]) -> Fx Patch Vector/36
  Body Contact 9/2(Fy patch [N]) -> Fy Patch Vector/36
  Fx Patch Vector/1 -> Net Fx at CoM/1
  Fy Patch Vector/1 -> Net Fy at CoM/1
  Net Fx at CoM/1 -> Fx_CoM [N]/1
  Net Fy at CoM/1 -> Fy_CoM [N]/1
  connections:
  Rigid Transform35/RConn1 -- Body Contact 33/LConn1
  Rigid Transform34/RConn1 -- Body Contact 32/LConn1
  Rigid Transform29/RConn1 -- Body Contact 25/LConn1
  Rigid Transform33/RConn1 -- Body Contact 31/LConn1
  Rigid Transform30/RConn1 -- Body Contact 28/LConn1
  Rigid Transform25/RConn1 -- Body Contact 24/LConn1
  Rigid Transform36/RConn1 -- Body Contact 34/LConn1
  Rigid Transform32/RConn1 -- Body Contact 30/LConn1
  Rigid Transform27/RConn1 -- Body Contact 26/LConn1
  Rigid Transform28/RConn1 -- Body Contact 27/LConn1
  Rigid Transform26/RConn1 -- Body Contact 35/LConn1
  Rigid Transform31/RConn1 -- Body Contact 29/LConn1
  Rigid Transform26/LConn1 -- CoM/RConn1 -- Rigid Transform6/LConn1 -- Rigid Transform5/LConn1 -- Rigid Transform4/LConn1 -- Rigid Transform3/LConn1 -- Rigid Transform2/LConn1 -- Rigid Transform1/LConn1 -- Rigid Transform7/LConn1 -- Rigid Transform8/LConn1 -- Rigid Transform9/LConn1 -- Rigid Transform10/LConn1 -- Rigid Transform11/LConn1 -- Rigid Transform12/LConn1 -- Rigid Transform17/LConn1 -- Rigid Transform13/LConn1 -- Rigid Transform18/LConn1 -- Rigid Transform19/LConn1 -- Rigid Transform20/LConn1 -- Rigid Transform21/LConn1 -- Rigid Transform22/LConn1 -- Rigid Transform23/LConn1 -- Rigid Transform24/LConn1 -- Rigid Transform15/LConn1 -- Rigid Transform16/LConn1 -- Rigid Transform14/LConn1 -- Rigid Transform29/LConn1 -- Rigid Transform25/LConn1 -- Rigid Transform30/LConn1 -- Rigid Transform31/LConn1 -- Rigid Transform32/LConn1 -- Rigid Transform33/LConn1 -- Rigid Transform34/LConn1 -- Rigid Transform35/LConn1 -- Rigid Transform36/LConn1 -- Rigid Transform27/LConn1 -- Rigid Transform28/LConn1
  Rigid Transform23/RConn1 -- Body Contact 21/LConn1
  Rigid Transform22/RConn1 -- Body Contact 20/LConn1
  Rigid Transform17/RConn1 -- Body Contact 13/LConn1
  Rigid Transform21/RConn1 -- Body Contact 19/LConn1
  Rigid Transform18/RConn1 -- Body Contact 16/LConn1
  Rigid Transform13/RConn1 -- Body Contact 12/LConn1
  Rigid Transform24/RConn1 -- Body Contact 22/LConn1
  Rigid Transform20/RConn1 -- Body Contact 18/LConn1
  Rigid Transform15/RConn1 -- Body Contact 14/LConn1
  Rigid Transform16/RConn1 -- Body Contact 15/LConn1
  Rigid Transform14/RConn1 -- Body Contact 23/LConn1
  Rigid Transform19/RConn1 -- Body Contact 17/LConn1
  Rigid Transform2/RConn1 -- Body Contact 1/LConn1
  Rigid Transform3/RConn1 -- Body Contact 2/LConn1
  Rigid Transform5/RConn1 -- Body Contact 4/LConn1
  Rigid Transform12/RConn1 -- Body Contact 11/LConn1
  Rigid Transform6/RConn1 -- Body Contact 5/LConn1
  Rigid Transform9/RConn1 -- Body Contact 8/LConn1
  Rigid Transform4/RConn1 -- Body Contact 3/LConn1
  Rigid Transform1/RConn1 -- "Body Contact "/LConn1
  Rigid Transform8/RConn1 -- Body Contact 7/LConn1
  Rigid Transform10/RConn1 -- Body Contact 9/LConn1
  Rigid Transform7/RConn1 -- Body Contact 6/LConn1
  Rigid Transform11/RConn1 -- Body Contact 10/LConn1

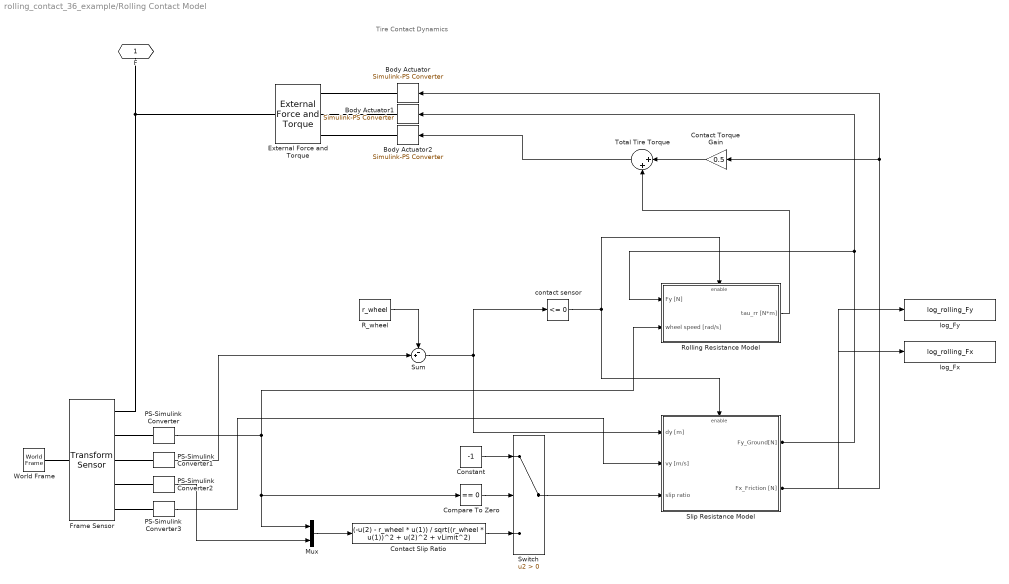
== system rolling_contact_36_example/Rolling Contact Model ==
  note: Tire Contact Dynamics
  " Body Actuator" : nesl_utility/Simulink-PS Converter  PhysicalDomain=network_engine_domain  SubClassName=ps_input  LeftPortType=input  RightPortType=output  PseudoPeriodic=off  Frequencies=[]  NoiseDistribution=none  NoiseParameters=[]  Unit=N  AffineConversion=off  FilteringAndDerivatives=zero  SimscapeFilterOrder=1  InputFilterTimeConstant=.001  UdotUserProvided=0
  " Body Actuator1" : nesl_utility/Simulink-PS Converter  PhysicalDomain=network_engine_domain  SubClassName=ps_input  LeftPortType=input  RightPortType=output  PseudoPeriodic=off  Frequencies=[]  NoiseDistribution=none  NoiseParameters=[]  Unit=N  AffineConversion=off  FilteringAndDerivatives=zero  SimscapeFilterOrder=1  InputFilterTimeConstant=.001  UdotUserProvided=0
  " Body Actuator2" : nesl_utility/Simulink-PS Converter  PhysicalDomain=network_engine_domain  SubClassName=ps_input  LeftPortType=input  RightPortType=output  PseudoPeriodic=off  Frequencies=[]  NoiseDistribution=none  NoiseParameters=[]  Unit=N*m  AffineConversion=off  FilteringAndDerivatives=zero  SimscapeFilterOrder=1  InputFilterTimeConstant=.001  UdotUserProvided=0
  Compare To Zero : simulink/Logic and Bit Operations/Compare To Zero  relop===  OutDataTypeStr=boolean
  Constant : Constant  Value=-1
  Contact Slip Ratio : Fcn  Expr=(-u(2) - r_wheel * u(1)) / sqrt((r_wheel * u(1))^2 + u(2)^2 + vLimit^2)
  Contact Torque Gain : Gain  Gain=0.5
  External Force and Torque : sm_lib/Forces and Torques/External Force and Torque  EnableForceX=on  EnableForceY=on  EnableForceZ=off  EnableForce=off  ForceResolutionFrame=World  EnableTorqueX=off  EnableTorqueY=off  EnableTorqueZ=on  EnableTorque=off  TorqueResolutionFrame=AttachedFrame
  Frame Sensor : sm_lib/Frames and Transforms/Transform Sensor  ObservationFrame=World  ExpressedInFrame=World  RotationSequence=XYX  SenseAngle=off  SenseAxis=off  SenseQ=off  SenseR=off  SenseRotationSequence=off  SenseOmegaX=off  SenseOmegaY=off  SenseOmegaZ=on  SenseOmega=off  SenseQDot=off  SenseRDot=off  SenseRotationSequenceDot=off  SenseAlphaX=off  SenseAlphaY=off  SenseAlphaZ=off  SenseAlpha=off  SenseQDDot=off  SenseRDDot=off  SenseX=off  SenseY=on  SenseZ=off  SenseXYZ=off  SenseRad=off  SenseAzim=off  SenseDist=off  SenseInc=off  SenseXDot=on  SenseYDot=on  SenseZDot=off  SenseXYZDot=off  SenseRadDot=off  SenseAzimDot=off  SenseDistDot=off  SenseIncDot=off  SenseXDDot=off  SenseYDDot=off  SenseZDDot=off  SenseXYZDDot=off  SenseRadDDot=off  SenseAzimDDot=off  SenseDistDDot=off  SenseIncDDot=off
  Mux : Mux  Inputs=2
  PS-Simulink Converter : nesl_utility/PS-Simulink Converter  PhysicalDomain=network_engine_domain  SubClassName=ps_output  LeftPortType=input  RightPortType=output  PseudoPeriodic=off  Frequencies=[]  VectorFormat=1-D array  Unit=rad/s  AffineConversion=off
  PS-Simulink Converter1 : nesl_utility/PS-Simulink Converter  PhysicalDomain=network_engine_domain  SubClassName=ps_output  LeftPortType=input  RightPortType=output  PseudoPeriodic=off  Frequencies=[]  VectorFormat=1-D array  Unit=m  AffineConversion=off
  PS-Simulink Converter2 : nesl_utility/PS-Simulink Converter  PhysicalDomain=network_engine_domain  SubClassName=ps_output  LeftPortType=input  RightPortType=output  PseudoPeriodic=off  Frequencies=[]  VectorFormat=1-D array  Unit=m/s  AffineConversion=off
  PS-Simulink Converter3 : nesl_utility/PS-Simulink Converter  PhysicalDomain=network_engine_domain  SubClassName=ps_output  LeftPortType=input  RightPortType=output  PseudoPeriodic=off  Frequencies=[]  VectorFormat=1-D array  Unit=m/s  AffineConversion=off
  R_wheel : Constant  Value=r_wheel
  Rolling Resistance Model : Subsystem
  Slip Resistance Model : Subsystem
  Sum : Sum  Inputs=-+|
  Switch : Switch  Criteria=u2 > Threshold  SaturateOnIntegerOverflow=off  InputSameDT=off
  Total Tire Torque : Sum  Inputs=|++
  World Frame : sm_lib/Frames and Transforms/World Frame
  contact sensor : simulink/Logic and Bit Operations/Compare To Zero  relop=<=  OutDataTypeStr=boolean
  log_Fx : ToWorkspace  VariableName=log_rolling_Fx  SaveFormat=Timeseries  SampleTime=-1
  log_Fy : ToWorkspace  VariableName=log_rolling_Fy  SaveFormat=Timeseries  SampleTime=-1
  F : PMIOPort  Side=Left
  wires:
  R_wheel/1 -> Sum/1
  Sum/1 -> contact sensor/1, Slip Resistance Model/1(dy [m])
  PS-Simulink Converter/1 -> Rolling Resistance Model/2(wheel speed [rad/s]), Mux/1, Compare To Zero/1
  Mux/1 -> Contact Slip Ratio/1
  PS-Simulink Converter1/1 -> Sum/2
  PS-Simulink Converter2/1 -> Mux/2
  Slip Resistance Model/1(Fy_Ground[N]) -> Rolling Resistance Model/1(Fy [N]), " Body Actuator1"/1, log_Fy/1
  Slip Resistance Model/2(Fx_Friction [N]) -> Contact Torque Gain/1, " Body Actuator"/1, log_Fx/1
  contact sensor/1 -> Slip Resistance Model/Enable, Rolling Resistance Model/Enable
  PS-Simulink Converter3/1 -> Slip Resistance Model/2(vy [m/s])
  Switch/1 -> Slip Resistance Model/3(slip ratio)
  Contact Slip Ratio/1 -> Switch/3
  Compare To Zero/1 -> Switch/2
  Constant/1 -> Switch/1
  Contact Torque Gain/1 -> Total Tire Torque/1
  Total Tire Torque/1 -> " Body Actuator2"/1
  Rolling Resistance Model/1(tau_rr [N*m]) -> Total Tire Torque/2
  connections:
  External Force and Torque/LConn1 -- " Body Actuator"/RConn1
  " Body Actuator1"/RConn1 -- External Force and Torque/LConn2
  F/RConn1 -- Frame Sensor/RConn1 -- External Force and Torque/RConn1
  PS-Simulink Converter3/LConn1 -- Frame Sensor/RConn5
  Frame Sensor/RConn2 -- PS-Simulink Converter/LConn1
  PS-Simulink Converter1/LConn1 -- Frame Sensor/RConn3
  PS-Simulink Converter2/LConn1 -- Frame Sensor/RConn4
  World Frame/RConn1 -- Frame Sensor/LConn1
  " Body Actuator2"/RConn1 -- External Force and Torque/LConn3

== system rolling_contact_36_example/36-Point Sliding Contact Model/Body Contact  ==
  note: Planar Ground Interaction Model
  " Body Actuator" : nesl_utility/Simulink-PS Converter  PhysicalDomain=network_engine_domain  SubClassName=ps_input  LeftPortType=input  RightPortType=output  PseudoPeriodic=off  Frequencies=[]  NoiseDistribution=none  NoiseParameters=[]  Unit=N  AffineConversion=off  FilteringAndDerivatives=zero  SimscapeFilterOrder=1  InputFilterTimeConstant=.001  UdotUserProvided=0
  " Body Actuator1" : nesl_utility/Simulink-PS Converter  PhysicalDomain=network_engine_domain  SubClassName=ps_input  LeftPortType=input  RightPortType=output  PseudoPeriodic=off  Frequencies=[]  NoiseDistribution=none  NoiseParameters=[]  Unit=N  AffineConversion=off  FilteringAndDerivatives=zero  SimscapeFilterOrder=1  InputFilterTimeConstant=.001  UdotUserProvided=0
  External Force and Torque : sm_lib/Forces and Torques/External Force and Torque  EnableForceX=on  EnableForceY=on  EnableForceZ=off  EnableForce=off  ForceResolutionFrame=World  EnableTorqueX=off  EnableTorqueY=off  EnableTorqueZ=off  EnableTorque=off  TorqueResolutionFrame=AttachedFrame
  Frame Sensor : sm_lib/Frames and Transforms/Transform Sensor  ObservationFrame=World  ExpressedInFrame=World  RotationSequence=XYX  SenseAngle=off  SenseAxis=off  SenseQ=off  SenseR=off  SenseRotationSequence=off  SenseOmegaX=off  SenseOmegaY=off  SenseOmegaZ=off  SenseOmega=off  SenseQDot=off  SenseRDot=off  SenseRotationSequenceDot=off  SenseAlphaX=off  SenseAlphaY=off  SenseAlphaZ=off  SenseAlpha=off  SenseQDDot=off  SenseRDDot=off  SenseX=on  SenseY=on  SenseZ=off  SenseXYZ=off  SenseRad=off  SenseAzim=off  SenseDist=off  SenseInc=off  SenseXDot=on  SenseYDot=on  SenseZDot=off  SenseXYZDot=off  SenseRadDot=off  SenseAzimDot=off  SenseDistDot=off  SenseIncDot=off  SenseXDDot=off  SenseYDDot=off  SenseZDDot=off  SenseXYZDDot=off  SenseRadDDot=off  SenseAzimDDot=off  SenseDistDDot=off  SenseIncDDot=off
  Ground Friction Model : Subsystem
  PS-Simulink Converter : nesl_utility/PS-Simulink Converter  PhysicalDomain=network_engine_domain  SubClassName=ps_output  LeftPortType=input  RightPortType=output  PseudoPeriodic=off  Frequencies=[]  VectorFormat=1-D array  Unit=m  AffineConversion=off
  PS-Simulink Converter1 : nesl_utility/PS-Simulink Converter  PhysicalDomain=network_engine_domain  SubClassName=ps_output  LeftPortType=input  RightPortType=output  PseudoPeriodic=off  Frequencies=[]  VectorFormat=1-D array  Unit=m  AffineConversion=off
  PS-Simulink Converter2 : nesl_utility/PS-Simulink Converter  PhysicalDomain=network_engine_domain  SubClassName=ps_output  LeftPortType=input  RightPortType=output  PseudoPeriodic=off  Frequencies=[]  VectorFormat=1-D array  Unit=m/s  AffineConversion=off
  PS-Simulink Converter3 : nesl_utility/PS-Simulink Converter  PhysicalDomain=network_engine_domain  SubClassName=ps_output  LeftPortType=input  RightPortType=output  PseudoPeriodic=off  Frequencies=[]  VectorFormat=1-D array  Unit=m/s  AffineConversion=off
  Sum : Sum  Inputs=-+|
  Terminator : Terminator
  World Frame : sm_lib/Frames and Transforms/World Frame
  contact sensor : simulink/Logic and Bit Operations/Compare To Zero  relop=<=  OutDataTypeStr=boolean
  yGround : Constant  Value=0
  F : PMIOPort  Side=Left
  Fx patch [N] : Outport
  Fy patch [N] : Outport  Port=2
  wires:
  Ground Friction Model/3(Stiction!) -> Terminator/1
  Ground Friction Model/2(Fx_Friction [N]) -> " Body Actuator"/1, Fx patch [N]/1
  Ground Friction Model/1(Fy_Ground[N]) -> " Body Actuator1"/1, Fy patch [N]/1
  contact sensor/1 -> Ground Friction Model/Enable
  yGround/1 -> Sum/1
  Sum/1 -> Ground Friction Model/1(dy [m]), contact sensor/1
  PS-Simulink Converter1/1 -> Sum/2
  PS-Simulink Converter3/1 -> Ground Friction Model/2(vy [m/s])
  PS-Simulink Converter/1 -> Ground Friction Model/3(x [m])
  PS-Simulink Converter2/1 -> Ground Friction Model/4(vx [m/s])
  connections:
  External Force and Torque/LConn1 -- " Body Actuator"/RConn1
  External Force and Torque/LConn2 -- " Body Actuator1"/RConn1
  F/RConn1 -- Frame Sensor/RConn1 -- External Force and Torque/RConn1
  PS-Simulink Converter3/LConn1 -- Frame Sensor/RConn5
  Frame Sensor/RConn2 -- PS-Simulink Converter/LConn1
  PS-Simulink Converter1/LConn1 -- Frame Sensor/RConn3
  PS-Simulink Converter2/LConn1 -- Frame Sensor/RConn4
  World Frame/RConn1 -- Frame Sensor/LConn1
